simulink model "FinalSolution_2025ElectricalComp"  (R2025b)
settings: Solver=VariableStepAuto  StartTime=0.0  StopTime=0.8  FixedStep=SPWM_Ts  RelTol=1e-3
InitFcn:
  | evalin(get_param(bdroot,'ModelWorkspace'),'eval(VF_InitializeCode);');
model workspace (MAT data in the model file):
  AC_LoadResistance = 9.23760430703
  AD_TimeConstant = 0.00025
  AD_a = [1 -0.881765205117]
  AD_b = [2.95586987209 -2.95586987209]
  CL_AAComp = 1.00249999972
  CL_AA_a = 0.998744152176
  CL_Kaw = 20
  CL_Ki = 1.6
  CL_Kp = 0.005
  CL_N = 200
  CL_Ts = 0.0001
  CL_Vref = 32
  CL_faa = 1000
  CL_fp = 50
  CL_mff = 0.94
  CL_mmax = 1
  CommonModeBias = 0.15
  CommonModeKp = 0.02
  CommonModeShift = 1
  ControlStartTime = 0.06
  DampingCapuF = 4.7
  DampingResistance = 30
  DeadtimeComp = 0.08
  DeadtimeCurrentBand = 0.2
  DutyFeedforward = 0
  DutyMax = 0.75
  FilterDCR = 0.3
  KiCurrentLoop = 5
  KiVoltageLoop = 5
  KpCurrentLoop = 0.08
  KpVoltageLoop = 0.2
  LoadConnectTime = 0.18
  MainFilterCapuF = 4.7
  PR_Gain = 1.25
  PR_a10 = [1 -1.99838562653 0.999372033695]
  PR_a11 = [1 -1.99817857535 0.999372066214]
  PR_a13 = [1 -1.99770539603 0.999372140529]
  PR_a16 = [1 -1.99684804391 0.99937227518]
  PR_a17 = [1 -1.99652293757 0.99937232624]
  PR_a19 = [1 -1.9958137982 0.999372437614]
  PR_a2 = [1 -1.99933241937 0.999371884997]
  PR_a4 = [1 -1.99921404574 0.999371903588]
  PR_a5 = [1 -1.99912527012 0.99937191753]
  PR_a7 = [1 -1.9988885544 0.999371954708]
  PR_a8 = [1 -1.99874062131 0.999371977941]
  PR_b10 = [0.236875635534 -0.472442728614 0.23556709308]
  PR_b11 = [0.215389811794 -0.429471148895 0.214081337101]
  PR_b13 = [0.182331988259 -0.363355656682 0.181023668423]
  PR_b16 = [0.148235597863 -0.295163156474 0.146927558611]
  PR_b17 = [0.139542977111 -0.277778021366 0.138235044255]
  PR_b19 = [0.124900915012 -0.248494129248 0.123593214235]
  PR_b2 = [0.425928775502 -0.847596177142 0.42166740164]
  PR_b4 = [0.279572378961 -0.55553023994 0.275957860979]
  PR_b5 = [0.246657018631 -0.490084248228 0.243427229597]
  PR_b7 = [0.202908225742 -0.403457656245 0.200549430503]
  PR_b8 = [0.186290317354 -0.370698545076 0.184408227722]
  PrechargeBypassTime = 0.16
  PrechargeResistance = 47
  RegenerativeMode = 1
  ReturnCurrent = 1.5
  ReturnRampTime = 0.08
  ReturnTs = 1e-05
  Return_Iref = 2
  SPWM_Ndead = 10
  SPWM_Tdead = 2e-06
  SPWM_Ts = 2e-07
  SPWM_Vgate = 10
  SPWM_f1 = 50
  SPWM_fs = 20000
  SPWM_m = 0.8
  Test_Mode = 1
  VF_CurrentN = 2000
  VF_CurrentRampTime = 0.1
  VF_InitializeCode = '% Executed in the adjustable model workspace by the embedded InitFcn.
% User settings: CL_Vref [line-line fundamental Vrms], SPWM_f1 [Hz], Return_Iref [line Arms].
assert(isscalar(SPWM_f1)&&isfinite(SPWM_f1)&&SPWM_f1>=20&&SPWM_f1<=100,''SPWM_f1 must be between 20 and 100 Hz.'');
assert(isscalar(CL_Vref)&&isfinite(CL_Vref)&&CL_Vref>0&&CL_Vref<=32,''CL_Vref must be greater than 0 and no more than 32 line-line Vrms. Low-voltage regenerative operation requires separate validation.'');
assert(isscalar(Return_Iref)&&isfinite(Return_Iref)&&Return_Iref>=0&&Return_Iref<=2,''Return_Iref must be between 0 and 2 line Arms.'');
assert(isscalar(VF_CurrentRampTime)&&isfinite(VF_CurrentRampTime)&&VF_CurrentRampTime>0,''VF_CurrentRampTime must be positive.'');
CL_N=round(1/(SPWM_f1*CL_Ts));
VF_CurrentN=round(1/(SPWM_f1*ReturnTs));
VF_ReturnStart=max(0.08,2/SPWM_f1);
CL_AA_a=exp(-2*pi*CL_faa*SPWM_Ts);
CL_AAComp=((1-CL_AA_a)^2+2*CL_AA_a*(1-cos(2*pi*SPWM_f1*SPWM_Ts)))/(1-CL_AA_a)^2;
CL_mff=min(CL_mmax,VF_mff32*CL_Vref/32);
% Preserve the original coefficients exactly at 50 Hz. At other frequencies,
% shift the analog resonances, retaining their original damping and s terms.
vf_harmonics=[2 4 5 7 8 10 11 13 16 17 19];
vf_k=2/ReturnTs;
for vf_h=vf_harmonics
    vf_bn=sprintf(''b%d'',vf_h);vf_an=sprintf(''a%d'',vf_h);
    if SPWM_f1==50
        vf_b=VF_PR_Base50.(vf_bn);vf_a=VF_PR_Base50.(vf_an);
    else
        vf_ac=VF_PR_Analog50.(vf_an);vf_bc=VF_PR_Analog50.(vf_bn);
        vf_ratio=(SPWM_f1/50)^2;
        vf_ac(3)=vf_ac(3)*vf_ratio;
        vf_bc(3)=vf_bc(3)*vf_ratio;
        vf_a=[vf_ac(1)*vf_k^2+vf_ac(2)*vf_k+vf_ac(3),-2*vf_ac(1)*vf_k^2+2*vf_ac(3),vf_ac(1)*vf_k^2-vf_ac(2)*vf_k+vf_ac(3)];
        vf_b=[vf_bc(1)*vf_k^2+vf_bc(2)*vf_k+vf_bc(3),-2*vf_bc(1)*vf_k^2+2*vf_bc(3),vf_bc(1)*vf_k^2-vf_bc(2)*vf_k+vf_bc(3)];
        vf_b=vf_b/vf_a(1);vf_a=vf_a/vf_a(1);
    end
    eval(sprintf(''PR_b%d=vf_b;PR_a%d=vf_a;'',vf_h,vf_h));
end
clear vf_harmonics vf_k vf_h vf_bn vf_an vf_b vf_a vf_ac vf_bc vf_ratio

assert(isscalar(Test_Mode)&&any(Test_Mode==[0 1]),''Test_Mode must be 0 (resistive) or 1 (regenerative).'');
VF_LoadR=CL_Vref/(sqrt(3)*max(Return_Iref,1e-6));
'
  VF_LoadR = 9.23760430703
  VF_PR_Analog50.a2 = [1 62.8318530718 394784.176044]
  VF_PR_Analog50.b2 = [0.423935411387 426.275467004 5.55291384469e-07]
  VF_PR_Analog50.a4 = [1 62.8318530718 1579136.70417]
  VF_PR_Analog50.b4 = [0.277863348184 361.579621149 0]
  VF_PR_Analog50.a5 = [1 62.8318530718 2467401.10027]
  VF_PR_Analog50.b5 = [0.245134221798 323.100293186 5.55320147806e-07]
  VF_PR_Analog50.a7 = [1 62.8318530718 4836106.15653]
  VF_PR_Analog50.b7 = [0.201816592653 235.982146035 0]
  VF_PR_Analog50.a8 = [1 62.8318530718 6316546.8167]
  VF_PR_Analog50.b8 = [0.185436770913 188.297811498 0]
  VF_PR_Analog50.a10 = [1 62.8318530718 9869604.40109]
  VF_PR_Analog50.b10 = [0.236353860723 130.927641424 0]
  VF_PR_Analog50.a11 = [1 62.8318530718 11942221.3253]
  VF_PR_Analog50.b11 = [0.214867146112 130.927641424 0]
  VF_PR_Analog50.a13 = [1 62.8318530718 16679631.4378]
  VF_PR_Analog50.b13 = [0.181810662095 130.927641424 -2.77758691062e-07]
  VF_PR_Analog50.a16 = [1 62.8318530718 25266187.2668]
  VF_PR_Analog50.b16 = [0.147721162952 130.927641424 0]
  VF_PR_Analog50.a17 = [1 62.8318530718 28523156.7191]
  VF_PR_Analog50.b17 = [0.139031682778 130.927641424 0]
  VF_PR_Analog50.a19 = [1 62.8318530718 35629271.8879]
  VF_PR_Analog50.b19 = [0.124396768802 130.927641424 1.38945090303e-07]
  VF_PR_Base50.b2 = [0.425928775502 -0.847596177142 0.42166740164]
  VF_PR_Base50.a2 = [1 -1.99933241937 0.999371884997]
  VF_PR_Base50.b4 = [0.279572378961 -0.55553023994 0.275957860979]
  VF_PR_Base50.a4 = [1 -1.99921404574 0.999371903588]
  VF_PR_Base50.b5 = [0.246657018631 -0.490084248228 0.243427229597]
  VF_PR_Base50.a5 = [1 -1.99912527012 0.99937191753]
  VF_PR_Base50.b7 = [0.202908225742 -0.403457656245 0.200549430503]
  VF_PR_Base50.a7 = [1 -1.9988885544 0.999371954708]
  VF_PR_Base50.b8 = [0.186290317354 -0.370698545076 0.184408227722]
  VF_PR_Base50.a8 = [1 -1.99874062131 0.999371977941]
  VF_PR_Base50.b10 = [0.236875635534 -0.472442728614 0.23556709308]
  VF_PR_Base50.a10 = [1 -1.99838562653 0.999372033695]
  VF_PR_Base50.b11 = [0.215389811794 -0.429471148895 0.214081337101]
  VF_PR_Base50.a11 = [1 -1.99817857535 0.999372066214]
  VF_PR_Base50.b13 = [0.182331988259 -0.363355656682 0.181023668423]
  VF_PR_Base50.a13 = [1 -1.99770539603 0.999372140529]
  VF_PR_Base50.b16 = [0.148235597863 -0.295163156474 0.146927558611]
  VF_PR_Base50.a16 = [1 -1.99684804391 0.99937227518]
  VF_PR_Base50.b17 = [0.139542977111 -0.277778021366 0.138235044255]
  VF_PR_Base50.a17 = [1 -1.99652293757 0.99937232624]
  VF_PR_Base50.b19 = [0.124900915012 -0.248494129248 0.123593214235]
  VF_PR_Base50.a19 = [1 -1.9958137982 0.999372437614]
  VF_ReturnStart = 0.08
  VF_mff32 = 0.94
  VoltageRampRate = 100
  op_snapshot1 = opcond.OperatingPoint
  op_snapshot1.Model_ = 'boost'
  op_snapshot1.Time_ = 0.18
  op_snapshot1.States_(1) = opcond.StatePoint
  op_snapshot1.States_(1).Nx_ = 1
  op_snapshot1.States_(1).Block_ = 'boost/Capacitor'
  op_snapshot1.States_(1).StateName_ = 'boost.Capacitor.vc'
  op_snapshot1.States_(1).x_ = 58.5589398174
  op_snapshot1.States_(2) = opcond.StatePoint
  op_snapshot1.States_(2).Nx_ = 1
  op_snapshot1.States_(2).Block_ = 'boost/Capacitor1'
  op_snapshot1.States_(2).StateName_ = 'boost.Capacitor1.vc'
  op_snapshot1.States_(2).x_ = 58.5589398174
  op_snapshot1.States_(3) = opcond.StatePoint
  op_snapshot1.States_(3).Nx_ = 1
  op_snapshot1.States_(3).Block_ = 'boost/Capacitor1'
  op_snapshot1.States_(3).StateName_ = 'boost.Capacitor1.i'
  op_snapshot1.States_(3).x_ = 8.21038980487
  op_snapshot1.States_(4) = opcond.StatePoint
  op_snapshot1.States_(4).Nx_ = 1
  op_snapshot1.States_(4).Block_ = 'boost/Capacitor5'
  op_snapshot1.States_(4).StateName_ = 'boost.Capacitor5.vc'
  op_snapshot1.States_(4).x_ = 58.5589398174
  op_snapshot1.States_(5) = opcond.StatePoint
  op_snapshot1.States_(5).Nx_ = 1
  op_snapshot1.States_(5).Block_ = 'boost/Capacitor5'
  op_snapshot1.States_(5).StateName_ = 'boost.Capacitor5.i'
  op_snapshot1.States_(5).x_ = 8.21038980487
  op_snapshot1.States_(6) = opcond.StatePoint
  op_snapshot1.States_(6).Nx_ = 1
  op_snapshot1.States_(6).Block_ = 'boost/Diode'
  op_snapshot1.States_(6).StateName_ = 'boost.Diode.private.Diode.threshold'
  op_snapshot1.States_(6).x_ = 17.0081155809
  op_snapshot1.States_(7) = opcond.StatePoint
  op_snapshot1.States_(7).Nx_ = 1
  op_snapshot1.States_(7).Block_ = 'boost/Inductor1'
  op_snapshot1.States_(7).StateName_ = 'boost.Inductor1.i_L'
  op_snapshot1.States_(7).x_ = 0.585589085753
  op_snapshot1.States_(8) = opcond.StatePoint
  op_snapshot1.States_(8).Nx_ = 1
  op_snapshot1.States_(8).Block_ = 'boost/Inductor1'
  op_snapshot1.States_(8).StateName_ = 'boost.Inductor1.v'
  op_snapshot1.States_(8).x_ = 3.12421618864e-05
  op_snapshot1.States_(9) = opcond.StatePoint
  op_snapshot1.States_(9).Nx_ = 1
  op_snapshot1.States_(9).Block_ = 'boost/Inductor3'
  op_snapshot1.States_(9).StateName_ = 'boost.Inductor3.i_L'
  op_snapshot1.States_(9).x_ = 0.879083324239
  op_snapshot1.States_(10) = opcond.StatePoint
  op_snapshot1.States_(10).Nx_ = 1
  op_snapshot1.States_(10).Block_ = 'boost/Inductor3'
  op_snapshot1.States_(10).StateName_ = 'boost.Inductor3.v'
  op_snapshot1.States_(10).x_ = -26.1390098936
  op_snapshot1.States_(11) = opcond.StatePoint
  op_snapshot1.States_(11).Nx_ = 1
  op_snapshot1.States_(11).Block_ = 'boost/N-Channel MOSFET'
  op_snapshot1.States_(11).StateName_ = 'boost.N_Channel_MOSFET.capacitor_GD.vc'
  op_snapshot1.States_(11).x_ = -59.4226648146
  op_snapshot1.States_(12) = opcond.StatePoint
  op_snapshot1.States_(12).Nx_ = 1
  op_snapshot1.States_(12).Block_ = 'boost/N-Channel MOSFET'
  op_snapshot1.States_(12).StateName_ = 'boost.N_Channel_MOSFET.capacitor_GS.vc'
  op_snapshot1.States_(12).x_ = -5.94226648146e-15
  op_snapshot1.States_(13) = opcond.StatePoint
  op_snapshot1.States_(13).Nx_ = 1
  op_snapshot1.States_(13).Block_ = 'boost/N-Channel MOSFET'
  op_snapshot1.States_(13).StateName_ = 'boost.N_Channel_MOSFET.drainLeadRL.i'
  op_snapshot1.States_(13).x_ = -16.1290322888
  op_snapshot1.States_(14) = opcond.StatePoint
  op_snapshot1.States_(14).Nx_ = 1
  op_snapshot1.States_(14).Block_ = 'boost/N-Channel MOSFET'
  op_snapshot1.States_(14).StateName_ = 'boost.N_Channel_MOSFET.capacitor_GS.i'
  op_snapshot1.States_(14).x_ = 49504.950495
  op_snapshot1.States_(15) = opcond.StatePoint
  op_snapshot1.States_(15).Nx_ = 1
  op_snapshot1.States_(15).Block_ = 'boost/N-Channel MOSFET'
  op_snapshot1.States_(15).StateName_ = 'boost.N_Channel_MOSFET.mos.ids'
  op_snapshot1.States_(15).x_ = 5.94721697651e-11
  op_snapshot1.States_(16) = opcond.StatePoint
  op_snapshot1.States_(16).Nx_ = 1
  op_snapshot1.States_(16).Block_ = 'boost/PWM Generator/Carrier counter/Integrator with
    | Wrapped State
    | (Discrete or Continuous)/Discrete/Integrator'
  op_snapshot1.States_(16).x_ = 4.99999999998e-05
  op_snapshot1.States_(16).Ts_ = [1e-06 0]
  op_snapshot1.States_(16).SampleType_ = 'DSTATE'
  op_snapshot1.States_(17) = opcond.StatePoint
  op_snapshot1.States_(17).Nx_ = 1
  op_snapshot1.States_(17).Block_ = 'boost/PWM Generator/Carrier counter/Integrator with
    | Wrapped State
    | (Discrete or Continuous)1/Discrete/Integrator'
  op_snapshot1.States_(17).x_ = 9.99999999997e-05
  op_snapshot1.States_(17).Ts_ = [1e-06 0]
  op_snapshot1.States_(17).SampleType_ = 'DSTATE'
  op_snapshot1.States_(18) = opcond.StatePoint
  op_snapshot1.States_(18).Nx_ = 2
  op_snapshot1.States_(18).Block_ = 'boost/Simulink-PS Converter'
  op_snapshot1.States_(18).x_ = [0; 40]
  op_snapshot1.States_(18).SampleType_ = 'Discrete_3618734018'
  op_snapshot1.States_(19) = opcond.StatePoint
  op_snapshot1.States_(19).Nx_ = 2
  op_snapshot1.States_(19).Block_ = 'boost/Simulink-PS Converter1'
  op_snapshot1.States_(19).x_ = [1; 5]
  op_snapshot1.States_(19).Ts_ = {[0 0]; [1e-06 0]}
  op_snapshot1.States_(19).SampleType_ = 'Discrete_2417034514'
  op_snapshot1.States_(20) = opcond.StatePoint
  op_snapshot1.States_(20).Nx_ = 1
  op_snapshot1.States_(20).Block_ = 'boost/SoftSwitch/Capacitor2'
  op_snapshot1.States_(20).StateName_ = 'boost.SoftSwitch.Capacitor2.vc'
  op_snapshot1.States_(20).x_ = 39.9673344621
  op_snapshot1.States_(21) = opcond.StatePoint
  op_snapshot1.States_(21).Nx_ = 1
  op_snapshot1.States_(21).Block_ = 'boost/SoftSwitch/NPN Bipolar Transistor'
  op_snapshot1.States_(21).StateName_ = 'boost.SoftSwitch.NPN_Bipolar_Transistor.capacitor_be.vc'
  op_snapshot1.States_(21).x_ = 0.86898424391
  op_snapshot1.States_(22) = opcond.StatePoint
  op_snapshot1.States_(22).Nx_ = 1
  op_snapshot1.States_(22).Block_ = 'boost/SoftSwitch/NPN Bipolar Transistor'
  op_snapshot1.States_(22).StateName_ = 'boost.SoftSwitch.NPN_Bipolar_Transistor.capacitor_bc.vc'
  op_snapshot1.States_(22).x_ = 0.850383356077
  op_snapshot1.States_(23) = opcond.StatePoint
  op_snapshot1.States_(23).Nx_ = 1
  op_snapshot1.States_(23).Block_ = 'boost/SoftSwitch/NPN Bipolar Transistor'
  op_snapshot1.States_(23).StateName_ = 'boost.SoftSwitch.NPN_Bipolar_Transistor.collector_resistor.i'
  op_snapshot1.States_(23).x_ = 1.40646461747e-07
  op_snapshot1.States_(24) = opcond.StatePoint
  op_snapshot1.States_(24).Nx_ = 1
  op_snapshot1.States_(24).Block_ = 'boost/SoftSwitch/NPN Bipolar Transistor'
  op_snapshot1.States_(24).StateName_ = 'boost.SoftSwitch.NPN_Bipolar_Transistor.emitter_resistor.i'
  op_snapshot1.States_(24).x_ = -2.4450560899e-05
  op_snapshot1.States_(25) = opcond.StatePoint
  op_snapshot1.States_(25).Nx_ = 1
  op_snapshot1.States_(25).Block_ = 'boost/SoftSwitch/NPN Bipolar Transistor'
  op_snapshot1.States_(25).StateName_ = 'boost.SoftSwitch.NPN_Bipolar_Transistor.transistor.ic'
  op_snapshot1.States_(25).x_ = 1.40646462031e-07
  op_snapshot1.States_(26) = opcond.StatePoint
  op_snapshot1.States_(26).Nx_ = 1
  op_snapshot1.States_(26).Block_ = 'boost/SoftSwitch/NPN Bipolar Transistor'
  op_snapshot1.States_(26).StateName_ = 'boost.SoftSwitch.NPN_Bipolar_Transistor.transistor.ib'
  op_snapshot1.States_(26).x_ = 2.43099144448e-05
  op_snapshot1.States_(27) = opcond.StatePoint
  op_snapshot1.States_(27).Nx_ = 1
  op_snapshot1.States_(27).Block_ = 'boost/SoftSwitch/P-Channel MOSFET'
  op_snapshot1.States_(27).StateName_ = 'boost.SoftSwitch.P_Channel_MOSFET.capacitor_GD.vc'
  op_snapshot1.States_(27).x_ = -38.0984898932
  op_snapshot1.States_(28) = opcond.StatePoint
  op_snapshot1.States_(28).Nx_ = 1
  op_snapshot1.States_(28).Block_ = 'boost/SoftSwitch/P-Channel MOSFET'
  op_snapshot1.States_(28).StateName_ = 'boost.SoftSwitch.P_Channel_MOSFET.capacitor_GS.vc'
  op_snapshot1.States_(28).x_ = -39.9672465538
  op_snapshot1.States_(29) = opcond.StatePoint
  op_snapshot1.States_(29).Nx_ = 1
  op_snapshot1.States_(29).Block_ = 'boost/SoftSwitch/P-Channel MOSFET'
  op_snapshot1.States_(29).StateName_ = 'boost.SoftSwitch.P_Channel_MOSFET.capacitor_GS.i'
  op_snapshot1.States_(29).x_ = -2.82857431713e-11
  op_snapshot1.States_(30) = opcond.StatePoint
  op_snapshot1.States_(30).Nx_ = 1
  op_snapshot1.States_(30).Block_ = 'boost/SoftSwitch/P-Channel MOSFET'
  op_snapshot1.States_(30).StateName_ = 'boost.SoftSwitch.P_Channel_MOSFET.mos.ids'
  op_snapshot1.States_(30).x_ = -0.879083414389
  op_snapshot1.States_(31) = opcond.StatePoint
  op_snapshot1.States_(31).Nx_ = 2
  op_snapshot1.States_(31).Block_ = 'boost/SoftSwitch/Simulink-PS Converter3'
  op_snapshot1.States_(31).x_ = [0; 3.3]
  op_snapshot1.States_(31).Ts_ = {[0 0]; [0 1]}
  op_snapshot1.States_(31).SampleType_ = 'Discrete_2909875362'
  testadd = 0
undefined symbols (not defined in the file): DiscIntNeverNeededParam, dspblkCoreblockFVToolHelper, gcbh
libraries: fl_lib x37, ee_lib x37, nesl_utility x32
(part 1 of 4)
settings Model: Creator=liuhaobo  LastModifiedBy=liuhaobo
settings DataIOCC: SaveOutput=off  SignalLogging=off  SaveTime=off

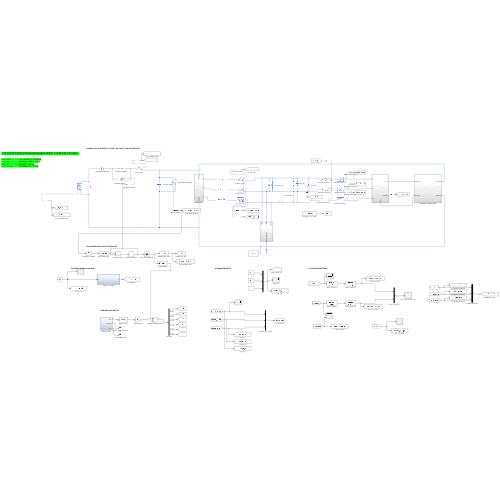
[thumbnail: Simulink's stored preview of the top-level diagram]
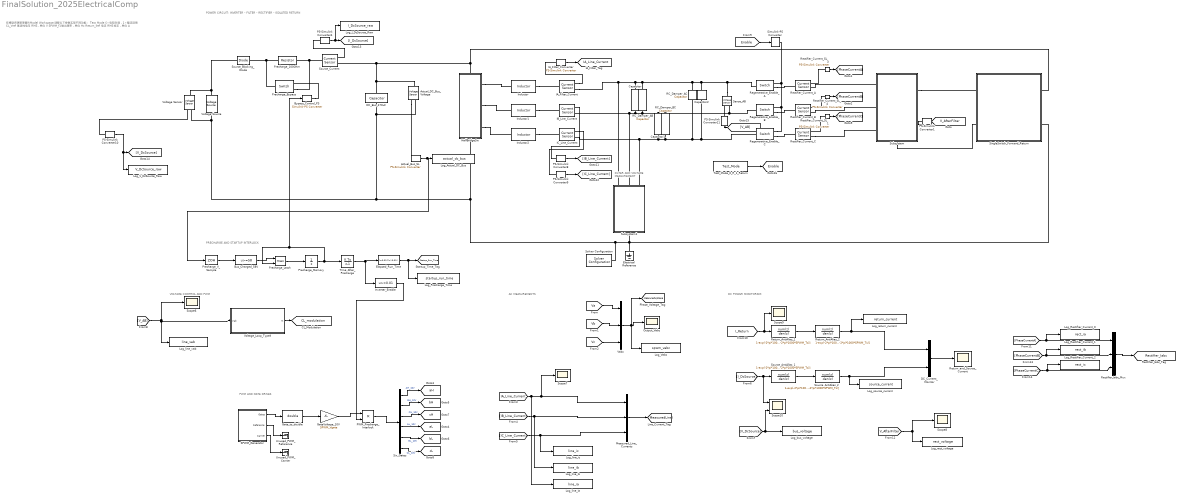
== system FinalSolution_2025ElectricalComp ==
  note: 在模型资源管理器的Model Workspace,调整以下参数实现不同功能：
      |
      | Test_Mode 0＝电阻负载，1＝整流回馈
      | CL_Vref 基波线电压 RMS，单位 V
      | SPWM_f1 输出频率，单位 Hz
      | Return_Iref 电流 RMS 给定，单位 A
      |
      | ​
      |
      | ​
      |
      | ​
      | ​
      | ​
      |
      | ​
      | ​
      | ​
      |
      | ​
      | ​
      | ​
  note: FILTER AND VOLTAGE MEASUREMENT
  note: PWM AND GATE DRIVES
  note: DC POWER MONITORING
  note: AC MEASUREMENTS
  note: VOLTAGE CONTROL AND PWM
  note: PRECHARGE AND STARTUP INTERLOCK
  note: POWER CIRCUIT: INVERTER - FILTER - RECTIFIER - ISOLATED RETURN
  Actual_Bus_SL : nesl_utility/PS-Simulink Converter  PhysicalDomain=network_engine_domain  SubClassName=ps_output  LeftPortType=input  RightPortType=output  PseudoPeriodic=off  Frequencies=[]  VectorFormat=inherit  Unit=inherit  AffineConversion=off
  Actual_DC_Bus_Voltage : fl_lib/Electrical/Electrical Sensors/Voltage Sensor
  Bus_Charged_58V : Fcn  Expr=u>=58
  Bypass_Control_PS : nesl_utility/Simulink-PS Converter  PhysicalDomain=network_engine_domain  SubClassName=ps_input  LeftPortType=input  RightPortType=output  PseudoPeriodic=off  Frequencies=[]  NoiseDistribution=none  NoiseParameters=[]  Unit=1  AffineConversion=off  FilteringAndDerivatives=provide  SimscapeFilterOrder=1  InputFilterTimeConstant=0.001  UdotUserProvided=0
  Capacitor : ee_lib/Passive/Capacitor  cap_option=ee.enum.passive.capacitor.capOption.const  c=MainFilterCapuF uF  Cvec=[1e-05, 1e-06] F  Vvec=[0, 10] V  CV_table_symmetry=ee.enum.passive.capacitor.tableSymmetry.yes  f_vec=[1, 10] kHz  DFext_vec=[.8, 1.2]  enable_C_tol=ee.enum.toleranceApplication.none  averaging_period=0 s  C_tol=5  tol_distribution=ee.enum.toleranceDistribution.uniform  nSigma=4  r=0.1 Ohm  g=0 1/Ohm  enable_operating_limits=ee.enum.enable.no  operating_limit_action=ee.enum.passive.reportOpLim.warn  max_working_voltage_range=[-25, 25] V  power_rating=1 W  maxTemperature=85 degC  thermalEnable=false  thermalMass=1 J/K  i_specify=off  i_priority=None  i=0 A  i_nominal_specify=off  i_nominal_value=1  i_nominal_unit=A  v_specify=off  v_priority=None  v=0 V  v_nominal_specify=off  v_nominal_value=1  v_nominal_unit=V  vc_specify=off  vc_priority=High  vc=0 V  vc_nominal_specify=off  vc_nominal_value=1  vc_nominal_unit=V  T_specify=off  T_priority=None  T=298.15 K  T_nominal_specify=off  T_nominal_value=1  T_nominal_unit=K
  Capacitor1 : ee_lib/Passive/Capacitor  cap_option=ee.enum.passive.capacitor.capOption.const  c=MainFilterCapuF uF  Cvec=[1e-05, 1e-06] F  Vvec=[0, 10] V  CV_table_symmetry=ee.enum.passive.capacitor.tableSymmetry.yes  f_vec=[1, 10] kHz  DFext_vec=[.8, 1.2]  enable_C_tol=ee.enum.toleranceApplication.none  averaging_period=0 s  C_tol=5  tol_distribution=ee.enum.toleranceDistribution.uniform  nSigma=4  r=0.1 Ohm  g=0 1/Ohm  enable_operating_limits=ee.enum.enable.no  operating_limit_action=ee.enum.passive.reportOpLim.warn  max_working_voltage_range=[-25, 25] V  power_rating=1 W  maxTemperature=85 degC  thermalEnable=false  thermalMass=1 J/K  i_specify=off  i_priority=None  i=0 A  i_nominal_specify=off  i_nominal_value=1  i_nominal_unit=A  v_specify=off  v_priority=None  v=0 V  v_nominal_specify=off  v_nominal_value=1  v_nominal_unit=V  vc_specify=off  vc_priority=High  vc=0 V  vc_nominal_specify=off  vc_nominal_value=1  vc_nominal_unit=V  T_specify=off  T_priority=None  T=298.15 K  T_nominal_specify=off  T_nominal_value=1  T_nominal_unit=K
  Capacitor2 : ee_lib/Passive/Capacitor  cap_option=ee.enum.passive.capacitor.capOption.const  c=MainFilterCapuF uF  Cvec=[1e-05, 1e-06] F  Vvec=[0, 10] V  CV_table_symmetry=ee.enum.passive.capacitor.tableSymmetry.yes  f_vec=[1, 10] kHz  DFext_vec=[.8, 1.2]  enable_C_tol=ee.enum.toleranceApplication.none  averaging_period=0 s  C_tol=5  tol_distribution=ee.enum.toleranceDistribution.uniform  nSigma=4  r=0.1 Ohm  g=0 1/Ohm  enable_operating_limits=ee.enum.enable.no  operating_limit_action=ee.enum.passive.reportOpLim.warn  max_working_voltage_range=[-25, 25] V  power_rating=1 W  maxTemperature=85 degC  thermalEnable=false  thermalMass=1 J/K  i_specify=off  i_priority=None  i=0 A  i_nominal_specify=off  i_nominal_value=1  i_nominal_unit=A  v_specify=off  v_priority=None  v=0 V  v_nominal_specify=off  v_nominal_value=1  v_nominal_unit=V  vc_specify=off  vc_priority=High  vc=0 V  vc_nominal_specify=off  vc_nominal_value=1  vc_nominal_unit=V  T_specify=off  T_priority=None  T=298.15 K  T_nominal_specify=off  T_nominal_value=1  T_nominal_unit=K
  DC_Bus_470uF : ee_lib/Passive/Capacitor  cap_option=ee.enum.passive.capacitor.capOption.const  c=470 uF  Cvec=[1e-05, 1e-06] F  Vvec=[0, 10] V  CV_table_symmetry=ee.enum.passive.capacitor.tableSymmetry.yes  f_vec=[1, 10] kHz  DFext_vec=[.8, 1.2]  enable_C_tol=ee.enum.toleranceApplication.none  averaging_period=0 s  C_tol=5  tol_distribution=ee.enum.toleranceDistribution.uniform  nSigma=4  r=0.05 Ohm  g=0 1/Ohm  enable_operating_limits=ee.enum.enable.no  operating_limit_action=ee.enum.passive.reportOpLim.warn  max_working_voltage_range=[-25, 25] V  power_rating=1 W  maxTemperature=85 degC  thermalEnable=false  thermalMass=1 J/K  i_specify=off  i_priority=None  i=0 A  i_nominal_specify=off  i_nominal_value=1  i_nominal_unit=A  v_specify=off  v_priority=None  v=0 V  v_nominal_specify=off  v_nominal_value=1  v_nominal_unit=V  vc_specify=on  vc_priority=High  vc=0 V  vc_nominal_specify=off  vc_nominal_value=1  vc_nominal_unit=V  T_specify=off  T_priority=None  T=298.15 K  T_nominal_specify=off  T_nominal_value=1  T_nominal_unit=K
  DC_Current_Monitor : Mux  Inputs=2
  Elapsed_Run_Time : Fcn  Expr=(u-0.01)*(u>0.01)
  Electrical Reference : fl_lib/Electrical/Electrical Elements/Electrical Reference
  GateVoltage_10V : Gain  Gain=SPWM_Vgate
  Gate_to_double : DataTypeConversion  OutDataTypeStr=double  SaturateOnIntegerOverflow=off  RndMeth=Floor
  HalfBridgeSw : Subsystem
      settings: PortSchema="{\"entries\":[{\"content\":{\"sides\":[{\"content\":{},\"type\":\"ConnectorPlacement.EquallySpacedRectSide\",\"uuid\":\"ae75b3c9-dbe6-4001-a3f7-dc49c66e7a48\"},{\"content\":{\"connectorIds\":[\"RConn1\",\"RConn2\",\"RConn3\"],\"side\":\"RIGHT\"},\"type\":\"ConnectorPlacement.EquallySpacedRectSide\",\"uuid\":\"9a154dca-401a-4e4a-9357-56ed3e6a572c\"},{\"content\":{\"connectorIds\":[\"LConn1\"],\"side\":\"TOP\"},\"type\":\"ConnectorPlacement.EquallySpacedRectSide\",\"uuid\":\"b8ce91a2-e6ab-44bc-8425-0a54f0d37f8f\"},{\"content\":{\"connectorIds\":[\"RConn4\"],\"side\":\"BOTTOM\"},\"type\":\"ConnectorPlacement.EquallySpacedRectSide\",\"uuid\":\"3bca5f9f-f47c-4c71-bd93-a8342182633e\"}]},\"type\":\"ConnectorPlacement.EquallySpacedConnector\",\"uuid\":\"6b9f288e-c97a-41ff-842b-17405c33e506\"}],\"packageUris\":[\"http://schema.mathworks.com/mf0/Connector/R2020b\"],\"version\":\"1.0\"}"
  IA_Filter_Converter : nesl_utility/PS-Simulink Converter  PhysicalDomain=network_engine_domain  SubClassName=ps_output  LeftPortType=input  RightPortType=output  PseudoPeriodic=off  Frequencies=[]  VectorFormat=inherit  Unit=inherit  AffineConversion=off
  IA_Filter_Current : fl_lib/Electrical/Electrical Sensors/Current Sensor
  IB_Line_Current : fl_lib/Electrical/Electrical Sensors/Current Sensor
  IC_Line_Current : fl_lib/Electrical/Electrical Sensors/Current Sensor
  Inductor : ee_lib/Passive/Inductor  l=680 uH  enable_L_tol=ee.enum.toleranceApplication.none  L_tol=20  tol_distribution=ee.enum.toleranceDistribution.uniform  nSigma=4  r=FilterDCR Ohm  g=1e-9 1/Ohm  enable_operating_limits=ee.enum.enable.no  operating_limit_action=ee.enum.passive.reportOpLim.warn  max_working_current=1 A  power_rating=1 W  i_L_specify=off  i_L_priority=High  i_L=0 A  i_L_nominal_specify=off  i_L_nominal_value=1  i_L_nominal_unit=A
  Inductor1 : ee_lib/Passive/Inductor  l=680 uH  enable_L_tol=ee.enum.toleranceApplication.none  L_tol=20  tol_distribution=ee.enum.toleranceDistribution.uniform  nSigma=4  r=FilterDCR Ohm  g=1e-9 1/Ohm  enable_operating_limits=ee.enum.enable.no  operating_limit_action=ee.enum.passive.reportOpLim.warn  max_working_current=1 A  power_rating=1 W  i_L_specify=off  i_L_priority=High  i_L=0 A  i_L_nominal_specify=off  i_L_nominal_value=1  i_L_nominal_unit=A
  Inductor2 : ee_lib/Passive/Inductor  l=680 uH  enable_L_tol=ee.enum.toleranceApplication.none  L_tol=20  tol_distribution=ee.enum.toleranceDistribution.uniform  nSigma=4  r=FilterDCR Ohm  g=1e-9 1/Ohm  enable_operating_limits=ee.enum.enable.no  operating_limit_action=ee.enum.passive.reportOpLim.warn  max_working_current=1 A  power_rating=1 W  i_L_specify=off  i_L_priority=High  i_L=0 A  i_L_nominal_specify=off  i_L_nominal_value=1  i_L_nominal_unit=A
  Inverter_Enable : Fcn  Expr=u>=0.01
  Log_Actual_DC_Bus : ToWorkspace  VariableName=actual_dc_bus  SaveFormat=Timeseries  SampleTime=2e-7
  Log_I_DcSource_Raw : ToWorkspace  VariableName=I_DcSource_raw  SaveFormat=Timeseries  SampleTime=2e-7
  Log_Precharge_Time : ToWorkspace  VariableName=startup_run_time  SaveFormat=Timeseries  SampleTime=1e-4
  Log_Rectifier_Current_0 : ToWorkspace  VariableName=rect_ia  SaveFormat=Timeseries  SampleTime=1e-5
  Log_Rectifier_Current_1 : ToWorkspace  VariableName=rect_ib  SaveFormat=Timeseries  SampleTime=1e-5
  Log_Rectifier_Current_2 : ToWorkspace  VariableName=rect_ic  SaveFormat=Timeseries  SampleTime=1e-5
  Log_V_DcSource_Raw : ToWorkspace  VariableName=V_DcSource_raw  SaveFormat=Timeseries  SampleTime=2e-7
  Log_Vabc : ToWorkspace  VariableName=spwm_vabc  SaveFormat=Timeseries  SampleTime=1e-5
  Log_bus_voltage : ToWorkspace  VariableName=bus_voltage  SaveFormat=Timeseries  SampleTime=1e-5
  Log_line_ia : ToWorkspace  VariableName=line_ia  SaveFormat=Timeseries  SampleTime=1e-5
  Log_line_ib : ToWorkspace  VariableName=line_ib  SaveFormat=Timeseries  SampleTime=1e-5
  Log_line_ic : ToWorkspace  VariableName=line_ic  SaveFormat=Timeseries  SampleTime=1e-5
  Log_line_vab : ToWorkspace  VariableName=line_vab  SaveFormat=Timeseries  SampleTime=1e-5
  Log_rect_voltage : ToWorkspace  VariableName=rect_voltage  SaveFormat=Timeseries  SampleTime=1e-5
  Log_return_current : ToWorkspace  VariableName=return_current  SaveFormat=Timeseries  SampleTime=1e-5
  Log_source_current : ToWorkspace  VariableName=source_current  SaveFormat=Timeseries  SampleTime=1e-5
  Measured_Line_Currents : Mux  Inputs=3
  Output_Vabc : Scope
      settings: TimeSpan=0.45  ActiveDisplayYMinimum=-33.890713785562866  ActiveDisplayYMaximum=29.13545276255644
  PS-Simulink Converter{1,4,8..11} (6 alike) : nesl_utility/PS-Simulink Converter  PhysicalDomain=network_engine_domain  SubClassName=ps_output  LeftPortType=input  RightPortType=output  PseudoPeriodic=off  Frequencies=[]  VectorFormat=inherit  Unit=inherit  AffineConversion=off
  PWM_Precharge_Interlock : Product  Inputs=**
  Precharge_100Ohm : ee_lib/Passive/Resistor  R=100 Ohm  enable_R_tol=ee.enum.toleranceApplication.none  R_tol=5  tol_distribution=ee.enum.toleranceDistribution.uniform  nSigma=4  enable_operating_limits=ee.enum.enable.no  operating_limit_action=ee.enum.passive.reportOpLim.warn  power_rating=1 W  max_working_voltage=100 V  noise_mode=ee.enum.sources.noise.Disabled  Tdevice=25 degC  sample_time=1e-3 s  repeatability=ee.enum.ic.repeatability.notRepeatable  user_seed=0  auto_seed=846339619  power_derating_T1=70 degC  power_derating_T2=155 degC  operating_temperature_range_vec=[-50, 150] degC  alpha=3.93e-3 1/K  Tmeas=25 degC  thermal_mass=100 J/K  temperature_specify=off  temperature_priority=High  temperature=298.15 K  temperature_nominal_specify=off  temperature_nominal_value=1  temperature_nominal_unit=K
  Precharge_Bypass : fl_lib/Electrical/Electrical Elements/Switch  R_closed=0.01 Ohm  G_open=1e-8 1/Ohm  Threshold=0.5  i_specify=off  i_priority=None  i=0 A  i_nominal_specify=off  i_nominal_value=1  i_nominal_unit=A  v_specify=off  v_priority=None  v=0 V  v_nominal_specify=off  v_nominal_value=1  v_nominal_unit=V
  Precharge_Latch : MinMax  Function=max  Inputs=2
  Precharge_Memory : UnitDelay  SampleTime=1e-4  HasFrameUpgradeWarning=on
  Precharge_V_Sample : ZeroOrderHold  SampleTime=1e-4
  RC_Damper_AB : ee_lib/Passive/Capacitor  cap_option=ee.enum.passive.capacitor.capOption.const  c=DampingCapuF uF  Cvec=[1e-05, 1e-06] F  Vvec=[0, 10] V  CV_table_symmetry=ee.enum.passive.capacitor.tableSymmetry.yes  f_vec=[1, 10] kHz  DFext_vec=[.8, 1.2]  enable_C_tol=ee.enum.toleranceApplication.none  averaging_period=0 s  C_tol=5  tol_distribution=ee.enum.toleranceDistribution.uniform  nSigma=4  r=DampingResistance Ohm  g=0 1/Ohm  enable_operating_limits=ee.enum.enable.no  operating_limit_action=ee.enum.passive.reportOpLim.warn  max_working_voltage_range=[-25, 25] V  power_rating=1 W  maxTemperature=85 degC  thermalEnable=false  thermalMass=1 J/K  i_specify=off  i_priority=None  i=0 A  i_nominal_specify=off  i_nominal_value=1  i_nominal_unit=A  v_specify=off  v_priority=None  v=0 V  v_nominal_specify=off  v_nominal_value=1  v_nominal_unit=V  vc_specify=off  vc_priority=High  vc=0 V  vc_nominal_specify=off  vc_nominal_value=1  vc_nominal_unit=V  T_specify=off  T_priority=None  T=298.15 K  T_nominal_specify=off  T_nominal_value=1  T_nominal_unit=K
  RC_Damper_AC : ee_lib/Passive/Capacitor  cap_option=ee.enum.passive.capacitor.capOption.const  c=DampingCapuF uF  Cvec=[1e-05, 1e-06] F  Vvec=[0, 10] V  CV_table_symmetry=ee.enum.passive.capacitor.tableSymmetry.yes  f_vec=[1, 10] kHz  DFext_vec=[.8, 1.2]  enable_C_tol=ee.enum.toleranceApplication.none  averaging_period=0 s  C_tol=5  tol_distribution=ee.enum.toleranceDistribution.uniform  nSigma=4  r=DampingResistance Ohm  g=0 1/Ohm  enable_operating_limits=ee.enum.enable.no  operating_limit_action=ee.enum.passive.reportOpLim.warn  max_working_voltage_range=[-25, 25] V  power_rating=1 W  maxTemperature=85 degC  thermalEnable=false  thermalMass=1 J/K  i_specify=off  i_priority=None  i=0 A  i_nominal_specify=off  i_nominal_value=1  i_nominal_unit=A  v_specify=off  v_priority=None  v=0 V  v_nominal_specify=off  v_nominal_value=1  v_nominal_unit=V  vc_specify=off  vc_priority=High  vc=0 V  vc_nominal_specify=off  vc_nominal_value=1  vc_nominal_unit=V  T_specify=off  T_priority=None  T=298.15 K  T_nominal_specify=off  T_nominal_value=1  T_nominal_unit=K
  RC_Damper_BC : ee_lib/Passive/Capacitor  cap_option=ee.enum.passive.capacitor.capOption.const  c=DampingCapuF uF  Cvec=[1e-05, 1e-06] F  Vvec=[0, 10] V  CV_table_symmetry=ee.enum.passive.capacitor.tableSymmetry.yes  f_vec=[1, 10] kHz  DFext_vec=[.8, 1.2]  enable_C_tol=ee.enum.toleranceApplication.none  averaging_period=0 s  C_tol=5  tol_distribution=ee.enum.toleranceDistribution.uniform  nSigma=4  r=DampingResistance Ohm  g=0 1/Ohm  enable_operating_limits=ee.enum.enable.no  operating_limit_action=ee.enum.passive.reportOpLim.warn  max_working_voltage_range=[-25, 25] V  power_rating=1 W  maxTemperature=85 degC  thermalEnable=false  thermalMass=1 J/K  i_specify=off  i_priority=None  i=0 A  i_nominal_specify=off  i_nominal_value=1  i_nominal_unit=A  v_specify=off  v_priority=None  v=0 V  v_nominal_specify=off  v_nominal_value=1  v_nominal_unit=V  vc_specify=off  vc_priority=High  vc=0 V  vc_nominal_specify=off  vc_nominal_value=1  vc_nominal_unit=V  T_specify=off  T_priority=None  T=298.15 K  T_nominal_specify=off  T_nominal_value=1  T_nominal_unit=K
  Rectifier_Current_A : fl_lib/Electrical/Electrical Sensors/Current Sensor
  Rectifier_Current_B : fl_lib/Electrical/Electrical Sensors/Current Sensor
  Rectifier_Current_C : fl_lib/Electrical/Electrical Sensors/Current Sensor
  Rectifier_Current_SL_1 : nesl_utility/PS-Simulink Converter  PhysicalDomain=network_engine_domain  SubClassName=ps_output  LeftPortType=input  RightPortType=output  PseudoPeriodic=off  Frequencies=[]  VectorFormat=inherit  Unit=inherit  AffineConversion=off
  Rectifier_Current_SL_3 : nesl_utility/PS-Simulink Converter  PhysicalDomain=network_engine_domain  SubClassName=ps_output  LeftPortType=input  RightPortType=output  PseudoPeriodic=off  Frequencies=[]  VectorFormat=inherit  Unit=inherit  AffineConversion=off
  Rectifier_Current_SL_4 : nesl_utility/PS-Simulink Converter  PhysicalDomain=network_engine_domain  SubClassName=ps_output  LeftPortType=input  RightPortType=output  PseudoPeriodic=off  Frequencies=[]  VectorFormat=inherit  Unit=inherit  AffineConversion=off
  Rectifier_Iabc_Mux : Mux  Inputs=3
  Regenerative_Enable_A : fl_lib/Electrical/Electrical Elements/Switch  R_closed=0.001 Ohm  G_open=1e-8 1/Ohm  Threshold=0.5  i_specify=off  i_priority=None  i=0 A  i_nominal_specify=off  i_nominal_value=1  i_nominal_unit=A  v_specify=off  v_priority=None  v=0 V  v_nominal_specify=off  v_nominal_value=1  v_nominal_unit=V
  Regenerative_Enable_B : fl_lib/Electrical/Electrical Elements/Switch  R_closed=0.001 Ohm  G_open=1e-8 1/Ohm  Threshold=0.5  i_specify=off  i_priority=None  i=0 A  i_nominal_specify=off  i_nominal_value=1  i_nominal_unit=A  v_specify=off  v_priority=None  v=0 V  v_nominal_specify=off  v_nominal_value=1  v_nominal_unit=V
  Regenerative_Enable_C : fl_lib/Electrical/Electrical Elements/Switch  R_closed=0.001 Ohm  G_open=1e-8 1/Ohm  Threshold=0.5  i_specify=off  i_priority=None  i=0 A  i_nominal_specify=off  i_nominal_value=1  i_nominal_unit=A  v_specify=off  v_priority=None  v=0 V  v_nominal_specify=off  v_nominal_value=1  v_nominal_unit=V
  Return_AntiAlias_1 : DiscreteTransferFcn  LoadFcn=dspblkCoreblockFVToolHelper(gcbh,'load');  Numerator=1-exp(-2*pi*1000*SPWM_Ts)  Denominator=[1 -exp(-2*pi*1000*SPWM_Ts)]  SampleTime=SPWM_Ts
      settings: CopyFcn=dspblkCoreblockFVToolHelper(gcbh,'copy');  DeleteFcn=dspblkCoreblockFVToolHelper(gcbh,'close');  ModelCloseFcn=dspblkCoreblockFVToolHelper(gcbh,'close');  PreSaveFcn=dspblkCoreblockFVToolHelper(gcbh,'presave');  PostSaveFcn=dspblkCoreblockFVToolHelper(gcbh,'postsave');  CloseFcn=dspblkCoreblockFVToolHelper(gcbh,'close');
  Return_AntiAlias_2 : DiscreteTransferFcn  LoadFcn=dspblkCoreblockFVToolHelper(gcbh,'load');  Numerator=1-exp(-2*pi*1000*SPWM_Ts)  Denominator=[1 -exp(-2*pi*1000*SPWM_Ts)]  SampleTime=SPWM_Ts
      settings: CopyFcn=dspblkCoreblockFVToolHelper(gcbh,'copy');  DeleteFcn=dspblkCoreblockFVToolHelper(gcbh,'close');  ModelCloseFcn=dspblkCoreblockFVToolHelper(gcbh,'close');  PreSaveFcn=dspblkCoreblockFVToolHelper(gcbh,'presave');  PostSaveFcn=dspblkCoreblockFVToolHelper(gcbh,'postsave');  CloseFcn=dspblkCoreblockFVToolHelper(gcbh,'close');
  Return_and_Source_Current : Scope
      settings: TimeSpan=0.45  ActiveDisplayYMinimum=-1.6318711686877323  ActiveDisplayYMaximum=13.840029161585569
  SPWM_Generator : Subsystem
  Scope10 : Scope  NumInputPorts=2
      settings: TimeSpan=0.45  ActiveDisplayYMinimum=1.5123517215294964  ActiveDisplayYMaximum=3.5125756951052041  DataLoggingVariableName=ScopeData13
  Scope{6..9} (4 alike) : Scope
      Scope6 settings: TimeSpan=0.45  ActiveDisplayYMinimum=-57.071191510992435  ActiveDisplayYMaximum=47.909792025708484  DataLoggingVariableName=ScopeData7
      Scope7 settings: TimeSpan=0.45  ActiveDisplayYMinimum=-2.2284949845346662  ActiveDisplayYMaximum=11.052432592326353  DataLoggingVariableName=ScopeData8
      Scope8 settings: TimeSpan=0.45  ActiveDisplayYMinimum=-6.4194281382968352  ActiveDisplayYMaximum=57.77435748610214  DataLoggingVariableName=ScopeData9
      Scope9 settings: TimeSpan=0.45  ActiveDisplayYMinimum=-0.64862139488560366  ActiveDisplayYMaximum=3.3373579603379793  DataLoggingVariableName=ScopeData10
  Sense_AB : fl_lib/Electrical/Electrical Sensors/Voltage Sensor
  Simulink-PS Converter : nesl_utility/Simulink-PS Converter  PhysicalDomain=network_engine_domain  SubClassName=ps_input  LeftPortType=input  RightPortType=output  PseudoPeriodic=off  Frequencies=[]  NoiseDistribution=none  NoiseParameters=[]  Unit=1  AffineConversion=off  FilteringAndDerivatives=provide  SimscapeFilterOrder=1  InputFilterTimeConstant=0.001  UdotUserProvided=0
  SingleSwitch_Forward_Return : Subsystem
  Six_Gates : Demux  Outputs=6
  Solver Configuration : nesl_utility/Solver Configuration  PhysicalDomain=network_engine_domain  SubClassName=solver  LeftPortType=input  RightPortType=generic  Tones=[]  Harmonics=[]  SimulateNoise=off  Profile=off  UseLocalSampling=off  EnableSwitchedLinearOptims=on  FrequencyDomain=off  UseCCode=off  RelTol=0.001  AbsTol=0.001  MinStep=1e-09  ToWorkspace=off  RevertToSquareIcSolve=off  NumHomotopyIterations=100  PhasorMode=off  PhasorModeNumHarmonics=1  ConsistencySolver=NEWTON_XTOL_AFTER_FTOL  IndexReductionMethod=DerivativeReplacement  DoDC=off  ResidualTolerance=1e-09  ConsistencyTolSource=GLOBAL  ConsistencyAbsTol=0.001  ConsistencyRelTol=0.001  ConsistencyTolFactor=0.001  UseLocalSolver=on  LocalSolverChoice=NE_BACKWARD_EULER_ADVANCER  ResolveIndetEquations=on  FunctionEvalNumThread=1  LocalSolverSampleTime=60*SPWM_Ts  DoFixedCost=off  MaxNonlinIter=3  MaxModeIter=2  ComputeImpulses=off  ImpulseIterations=2  LinearAlgebra=auto  LinearAlgebraNumThread=0  EquationFormulation=NE_TIME_EF  DelaysMemoryBudget=1024  AutomaticFiltering=on  FilteringTimeConstant=0.001  PartitionStorageMethod=AS_NEEDED  PartitionMemoryBudget=1024  PartitionMethod=ROBUST  MultibodyUseLocalSolver=off  MultibodyLocalSolverChoice=ODE1  MultibodyLocalSolverSampleTime=0.001
  Source_AntiAlias_1 : DiscreteTransferFcn  Numerator=1-exp(-2*pi*1000*SPWM_Ts)  Denominator=[1 -exp(-2*pi*1000*SPWM_Ts)]  SampleTime=SPWM_Ts
  Source_AntiAlias_2 : DiscreteTransferFcn  LoadFcn=dspblkCoreblockFVToolHelper(gcbh,'load');  Numerator=1-exp(-2*pi*1000*SPWM_Ts)  Denominator=[1 -exp(-2*pi*1000*SPWM_Ts)]  SampleTime=SPWM_Ts
      settings: CopyFcn=dspblkCoreblockFVToolHelper(gcbh,'copy');  DeleteFcn=dspblkCoreblockFVToolHelper(gcbh,'close');  ModelCloseFcn=dspblkCoreblockFVToolHelper(gcbh,'close');  PreSaveFcn=dspblkCoreblockFVToolHelper(gcbh,'presave');  PostSaveFcn=dspblkCoreblockFVToolHelper(gcbh,'postsave');  CloseFcn=dspblkCoreblockFVToolHelper(gcbh,'close');
  Source_Blocking_Diode : ee_lib/Semiconductors & Converters/Diode  ModelType=ee.enum.diode.modelType.pwl  TableType=ee.enum.diode.tableType.IfMat  IfMat=[.07, .12, .19, 1.75, 4.24, 7.32, 11.2; .16, .3, .72, 2.14, 5.02, 8.35, 13.12] A  VfMat=[.9, 1.15, 1.25, 1.5, 1.75, 2.17, 2.6, 2.85; .58, .68, .75, 1.1, 1.38, 1.77, 2.27, 2.7] V  TjVec=[25, 125] degC  VfVec=[.5, .7, .9, 1.3, 1.7, 2.1, 2.5] V  IfVec=[.1, .2, .5, 1, 2, 4, 7, 10] A  IrMat=[1e-06, 2e-06, 5e-06, 1e-05, 2.5e-05, 5e-05, .0001; 2e-06, 5e-06, 1e-05, 4e-05, 8e-05, .0002, .0005] A  VrMat=[10, 100, 200, 250, 300, 325, 350; 10, 70, 160, 220, 270, 300, 320] V  VrVec=[10, 20, 40, 50, 70, 80, 100] V  IrVec=[1e-06, 2e-06, 5e-06, 1e-05, 2e-05, 5e-05, .0001] A  Vf=0.6 V  Ron=0.3 Ohm  Goff=1e-8 S  prmExp=ee.enum.diode.expParam.useTwo  I12=[.0137, .545] A  V12=[.6, .7] V  RS=0 Ohm  Tmeas=298.15 K  IS=1e-12 A  ec=1  I1=0.0137 A  V1=0.6 V  N_series=1  N_parallel=1  ZenerEnable=false  Rz=0.3 Ohm  BV=inf V  C_param=ee.enum.diode.capParam.fixed  CJ=0 pF  CJ0=5 pF  Vvec=[.1, 10, 100] V  Cvec=[3.5, 1, .4] pF  VJ=1 V  Mgrad=0.5  FC=0.5  Q_param=ee.enum.diode.recoveryParam.off  iRM=-7.15 A  iF=4 A  didt=-750 A/us  trr_factor=3  trr=115 ns  Qrr=150 nA*s  Vr=-600 V  Ls=150 nH  Erec=0.03 J  TT=50 ns  tau=100 ns  T_param=ee.enum.diode.temperatureParam.off  Tdevice=298.15 K  I1_T2=0.245 A  V1_T2=0.5 V  IS_T2=1.25e-7 A  Tmeas2=125 degC  XTI_param=ee.enum.diode.xtiParam.pn  XTI=3  EG_param=ee.enum.diode.egapParam.material_si  EG=1.11 eV  dBVdT=0 V/K  enable_fault_input=simscape.enum.onoff.off  i_specify=off  i_priority=None  i=0 A  i_nominal_specify=off  i_nominal_value=1  i_nominal_unit=A  v_specify=off  v_priority=None  v=0 V  v_nominal_specify=off  v_nominal_value=1  v_nominal_unit=V  v_capacitor_specify=off  v_capacitor_priority=None  v_capacitor=0 V  v_capacitor_nominal_specify=off  v_capacitor_nominal_value=1  v_capacitor_nominal_unit=V  Qj_specify=off  Qj_priority=High  Qj=0 C  Qj_nominal_specify=off  Qj_nominal_value=1  Qj_nominal_unit=C  i_diode_specify=off  i_diode_priority=None  i_diode=0 A  i_diode_nominal_specify=off  i_diode_nominal_value=1  i_diode_nominal_unit=A  v_diode_specify=off  v_diode_priority=None  v_diode=0 V  v_diode_nominal_specify=off  v_diode_nominal_value=1  v_diode_nominal_unit=V  i_capacitor_specify=off  i_capacitor_priority=None  i_capacitor=0 A  i_capacitor_nominal_specify=off  i_capacitor_nominal_value=1  i_capacitor_nominal_unit=A  power_dissipated_specify=off  power_dissipated_priority=None  power_dissipated=0 W  power_dissipated_nominal_specify=off  power_dissipated_nominal_value=1  power_dissipated_nominal_unit=W  fidelity_level=ee.enum.diode.fidelity.includeChargeDyn  rec_loss_model=ee.enum.diode.reverseRecoveryModel.fixed  ErecVal=0 J  scaleWithIandV=true  ErecMat=zeros(2, 3) J  TjrecVec=[298.15, 398.15] K  IfrecVec=[.1, 1, 10] A  IrecVal=10 A  VrecVal=10 V  tFilter=1 / 1000 / 100 s  thermal_network_parameterization=ee.enum.thermalNetworkTopology.junctionCase  Rth=[0, 10] K/W  Rth_Cauer=[1, 3, 10] K/W  Rth_Foster=[.08, .14, .22, .16] K/W  thermal_mass_parameterization=ee.enum.thermalNetwork.timeconstant  thermal_mass=[0, 1] J/K  thermal_mass_Cauer=[.1, .3, 1] J/K  thermal_mass_Foster=[.001, .005, .05, .5] J/K  thermal_time_constant=[0, 10] s  thermal_time_constant_Cauer=[1, 3, 10] s  thermal_time_constant_Foster=[7e-05, .0007, .01, .08] s  thermal_mass_initial_temperatures=[25, 25] degC  thermal_mass_initial_temperatures_Cauer=[25, 25, 25] degC  junction_thermal_mass=0.01 J/K  Tvec_initial_Foster=[25, 25, 25, 25] degC  no_thermal_network=0  junction_temperature_specify=off  junction_temperature_priority=None  junction_temperature=25 degC  junction_temperature_nominal_specify=off  junction_temperature_nominal_value=1  junction_temperature_nominal_unit=degC
  Source_Current : fl_lib/Electrical/Electrical Sensors/Current Sensor
  Subsystem : Subsystem
      settings: PortSchema="{\"entries\":[{\"content\":{\"sides\":[{\"content\":{\"connectorIds\":[\"LConn1\",\"LConn2\",\"LConn3\"]},\"type\":\"ConnectorPlacement.EquallySpacedRectSide\",\"uuid\":\"9f766f04-6e40-4052-a5a9-a5e6f39ea711\"},{\"content\":{\"connectorIds\":[\"RConn1\",\"RConn2\"],\"side\":\"RIGHT\"},\"type\":\"ConnectorPlacement.EquallySpacedRectSide\",\"uuid\":\"63a1d40d-36cd-4a84-988e-2ce64017f724\"},{\"content\":{\"side\":\"TOP\"},\"type\":\"ConnectorPlacement.EquallySpacedRectSide\",\"uuid\":\"8fba4ab4-5a90-4e94-988c-7905b6ed2d27\"},{\"content\":{\"connectorIds\":[\"RConn3\"],\"side\":\"BOTTOM\"},\"type\":\"ConnectorPlacement.EquallySpacedRectSide\",\"uuid\":\"e2c9ea40-78b7-4b0c-96ad-6d2e4b286f52\"}]},\"type\":\"ConnectorPlacement.EquallySpacedConnector\",\"uuid\":\"d3a3b661-c5b2-4547-837c-b30226954994\"}],\"packageUris\":[\"http://schema.mathworks.com/mf0/Connector/R2020b\"],\"version\":\"1.0\"}"
  Subsystem1 : Subsystem
  Test_Mode_0_R_1_Return : Constant  Value=Test_Mode
  Time_After_Precharge : DiscreteIntegrator  SampleTime=1e-4  ICPrevOutput=DiscIntNeverNeededParam  ICPrevScaledInput=DiscIntNeverNeededParam
  Unused_PWM_Carrier : Terminator
  Unused_PWM_Reference : Terminator
  Vabc : Mux  Inputs=3
  Voltage Sensor : fl_lib/Electrical/Electrical Sensors/Voltage Sensor
  Voltage Source : ee_lib/Sources/Voltage Source  dc_voltage=60 V  ac_voltage=0 V  ac_shift=0 rad  ac_frequency=50 Hz  noise_mode=ee.enum.sources.noise.Disabled  PSD=0 V^2/Hz  sample_time=1e-3 s  repeatability=ee.enum.sources.repeatability.NotRepeatable  user_seed=0  auto_seed=3499211588  i_specify=off  i_priority=None  i=0 A  i_nominal_specify=off  i_nominal_value=1  i_nominal_unit=A  v_specify=off  v_priority=None  v=0 V  v_nominal_specify=off  v_nominal_value=1  v_nominal_unit=V
  Voltage_Loop_TypeII : Subsystem
  tag scope: CL_modulation=global, Enable=global, IA_Line_Current=global, MeasuredLineI=global, MeasuredVphase=global, Rectifier_Iabc=global, Startup_Run_Time=global, V_AfterFilter=global, aH=global, aL=global, bH=global, bL=global, cH=global, cL=global
  wires:
  [Vc] -> Vabc/3
  [Vb] -> Vabc/2
  [Va] -> Vabc/1
  [V_DcSource] -> Log_bus_voltage/1, Scope10/2
  Return_AntiAlias_1/1 -> Return_AntiAlias_2/1
  Source_AntiAlias_1/1 -> Source_AntiAlias_2/1
  Voltage_Loop_TypeII/1(m) -> [CL_modulation]
  [V_AfterFilter] -> Scope8/1, Log_rect_voltage/1
  [I_DcSource] -> Source_AntiAlias_1/1, Scope10/1
  Measured_Line_Currents/1 -> [MeasuredLineI]
  [IA_Line_Current] -> Measured_Line_Currents/1, Scope7/1, Log_line_ia/1
  [IB_Line_Current] -> Measured_Line_Currents/2, Log_line_ib/1
  [IC_Line_Current] -> Measured_Line_Currents/3, Log_line_ic/1
  Vabc/1 -> Output_Vabc/1, Log_Vabc/1, [MeasuredVphase]
  DC_Current_Monitor/1 -> Return_and_Source_Current/1
  Source_AntiAlias_2/1 -> DC_Current_Monitor/2, Log_source_current/1
  PS-Simulink Converter8/1 -> [IB_Line_Current]
  PS-Simulink Converter9/1 -> [IC_Line_Current]
  PS-Simulink Converter11/1 -> [V_AB]
  [I_Return] -> Scope9/1, Return_AntiAlias_1/1
  PS-Simulink Converter1/1 -> [V_AfterFilter]
  IA_Filter_Converter/1 -> [IA_Line_Current]
  Test_Mode_0_R_1_Return/1 -> [Enable]
  Rectifier_Iabc_Mux/1 -> [Rectifier_Iabc]
  [PhaseCurrentC] -> Rectifier_Iabc_Mux/3, Log_Rectifier_Current_2/1
  [PhaseCurrentB] -> Rectifier_Iabc_Mux/2, Log_Rectifier_Current_1/1
  [PhaseCurrentA] -> Rectifier_Iabc_Mux/1, Log_Rectifier_Current_0/1
  [Enable] -> Simulink-PS Converter/1
  SPWM_Generator/3(Carrier) -> Unused_PWM_Carrier/1
  SPWM_Generator/2(Reference) -> Unused_PWM_Reference/1
  PS-Simulink Converter10/1 -> [V_DcSource], Log_V_DcSource_Raw/1
  [V_AB] -> Voltage_Loop_TypeII/1(Vab), Log_line_vab/1, Scope6/1
  SPWM_Generator/1(Gates) -> Gate_to_double/1
  Return_AntiAlias_2/1 -> Log_return_current/1, DC_Current_Monitor/1
  PWM_Precharge_Interlock/1 -> Six_Gates/1
  Inverter_Enable/1 -> PWM_Precharge_Interlock/2
  Elapsed_Run_Time/1 -> [Startup_Run_Time], Log_Precharge_Time/1
  Time_After_Precharge/1 -> Elapsed_Run_Time/1, Inverter_Enable/1
  Precharge_Latch/1 -> Precharge_Memory/1
  Precharge_Memory/1 -> Bypass_Control_PS/1, Precharge_Latch/2, Time_After_Precharge/1
  Bus_Charged_58V/1 -> Precharge_Latch/1
  Precharge_V_Sample/1 -> Bus_Charged_58V/1
  Actual_Bus_SL/1 -> Precharge_V_Sample/1, Log_Actual_DC_Bus/1
  Gate_to_double/1 -> GateVoltage_10V/1
  PS-Simulink Converter4/1 -> Log_I_DcSource_Raw/1, [I_DcSource]
  Six_Gates/6 -> [cL]  "CL_10V"
  Six_Gates/5 -> [bL]  "BL_10V"
  Six_Gates/4 -> [aL]  "AL_10V"
  Six_Gates/3 -> [cH]  "CH_10V"
  Six_Gates/2 -> [bH]  "BH_10V"
  Six_Gates/1 -> [aH]  "AH_10V"
  GateVoltage_10V/1 -> PWM_Precharge_Interlock/1
  Rectifier_Current_SL_3/1 -> [PhaseCurrentA]
  Rectifier_Current_SL_4/1 -> [PhaseCurrentB]
  Rectifier_Current_SL_1/1 -> [PhaseCurrentC]
  connections:
  Inductor2/RConn1 -- IC_Line_Current/LConn1
  Inductor1/RConn1 -- IB_Line_Current/LConn1
  IB_Line_Current/RConn1 -- PS-Simulink Converter8/LConn1
  IC_Line_Current/RConn1 -- PS-Simulink Converter9/LConn1
  IA_Filter_Current/RConn1 -- IA_Filter_Converter/LConn1
  Inductor/RConn1 -- IA_Filter_Current/LConn1
  PS-Simulink Converter11/LConn1 -- Sense_AB/RConn1
  Regenerative_Enable_C/RConn2 -- Rectifier_Current_C/LConn1
  Regenerative_Enable_B/RConn2 -- Rectifier_Current_B/LConn1
  Regenerative_Enable_A/RConn2 -- Rectifier_Current_A/LConn1
  Regenerative_Enable_B/RConn1 -- Regenerative_Enable_C/RConn1 -- Simulink-PS Converter/RConn1 -- Regenerative_Enable_A/RConn1
  Capacitor1/RConn1 -- Subsystem1/LConn3 -- IC_Line_Current/RConn2 -- Regenerative_Enable_C/LConn1 -- Capacitor2/RConn1 -- RC_Damper_AC/RConn1 -- RC_Damper_BC/RConn1
  Rectifier_Current_SL_3/LConn1 -- Rectifier_Current_A/RConn1
  Rectifier_Current_B/RConn1 -- Rectifier_Current_SL_4/LConn1
  Rectifier_Current_SL_1/LConn1 -- Rectifier_Current_C/RConn1
  PS-Simulink Converter10/LConn1 -- Voltage Sensor/RConn1
  Voltage Sensor/LConn1 -- Source_Blocking_Diode/LConn1 -- Voltage Source/LConn1
  Rectifier_Current_C/RConn2 -- Subsystem/LConn3
  Rectifier_Current_B/RConn2 -- Subsystem/LConn2
  Rectifier_Current_A/RConn2 -- Subsystem/LConn1
  Sense_AB/LConn1 -- RC_Damper_AB/LConn1 -- IA_Filter_Current/RConn2 -- Subsystem1/LConn1 -- Capacitor/LConn1 -- RC_Damper_AC/LConn1 -- Capacitor2/LConn1 -- Regenerative_Enable_A/LConn1
  Regenerative_Enable_B/LConn1 -- RC_Damper_BC/LConn1 -- IB_Line_Current/RConn2 -- Subsystem1/LConn2 -- Capacitor/RConn1 -- RC_Damper_AB/RConn1 -- Capacitor1/LConn1 -- Sense_AB/RConn2
  HalfBridgeSw/RConn1 -- Inductor/LConn1
  HalfBridgeSw/RConn3 -- Inductor2/LConn1
  HalfBridgeSw/RConn2 -- Inductor1/LConn1
  Subsystem/RConn2 -- PS-Simulink Converter1/LConn1
  Subsystem/RConn1 -- SingleSwitch_Forward_Return/LConn1
  Subsystem/RConn3 -- SingleSwitch_Forward_Return/LConn2
  Precharge_Bypass/LConn1 -- Source_Blocking_Diode/RConn1 -- Precharge_100Ohm/LConn1
  Precharge_100Ohm/RConn1 -- Precharge_Bypass/RConn2 -- Source_Current/LConn1
  Bypass_Control_PS/RConn1 -- Precharge_Bypass/RConn1
  DC_Bus_470uF/LConn1 -- Actual_DC_Bus_Voltage/LConn1 -- HalfBridgeSw/LConn1 -- SingleSwitch_Forward_Return/RConn1 -- Source_Current/RConn2
  PS-Simulink Converter4/LConn1 -- Source_Current/RConn1
  Voltage Source/RConn1 -- Solver Configuration/RConn1 -- Subsystem1/RConn1 -- SingleSwitch_Forward_Return/RConn2 -- Electrical Reference/LConn1 -- HalfBridgeSw/RConn4 -- DC_Bus_470uF/RConn1 -- Actual_DC_Bus_Voltage/RConn2 -- Voltage Sensor/RConn2
  Actual_DC_Bus_Voltage/RConn1 -- Actual_Bus_SL/LConn1
